simulink model "HSBI_Pedelec_Model"  (R2021b)
settings: Solver=ode4  StartTime=0.0  StopTime=t_end  FixedStep=t_step  RelTol=1e-3
values from neighbouring files (symbols this model uses):
  alphaGPX = [0 0 0 1.42108547152e-15 -7.50851856107e-05 -0.00056616369873 -0.00139814962361 -0.00223013361289 -0.00306211451479 -0.00389802874828 -0.00474974145994 -0.00561331371735 ... (6687 elements, 6687x1)]    [GPX_Simulink_Profil.mat]    (also in HSBI_Pedelec_Analyse_2.m = double(profil.alphaGPX(:)))
  c_R = 0.006    [HSBI_Pedelec_Parameter.m]
  c_w_A = 0.60    (= 0.6)    [HSBI_Pedelec_Parameter.m]
  E_Batt_nom = 500    [HSBI_Pedelec_Parameter.m]
  eta_G = 0.90    (= 0.9)    [HSBI_Pedelec_Parameter.m]
  eta_M = 0.80    (= 0.8)    [HSBI_Pedelec_Parameter.m]
  g = 9.81    [HSBI_Pedelec_Parameter.m]
  i_1 = 8    [HSBI_Pedelec_Parameter.m]
  i_2 = 5    [HSBI_Pedelec_Parameter.m]
  m = 135    [HSBI_Pedelec_Parameter.m]
  M_M_max = 5    [HSBI_Pedelec_Parameter.m]
  omega_M_max = 115    [HSBI_Pedelec_Parameter.m]
  P_F = 100    [HSBI_Pedelec_Parameter.m]
  P_M_max = 500    [HSBI_Pedelec_Parameter.m]
  r = 0.35    [HSBI_Pedelec_Parameter.m]
  rho = 1.225    [HSBI_Pedelec_Parameter.m]
  sGPX = [0 10 20 30 40 50 60 70 80 90 100 110 ... (6687 elements, 6687x1)]    [GPX_Simulink_Profil.mat]    (also in HSBI_Pedelec_Analyse_2.m = double(profil.sGPX(:)))
  SoC_0 = 1.00    (= 1)    [HSBI_Pedelec_Parameter.m]
  v_0 = 0    [HSBI_Pedelec_Analyse_2.m]
  v_fade = 23    [HSBI_Pedelec_Parameter.m]
  v_gs = 15    [HSBI_Pedelec_Parameter.m]
  v_max = 25    [HSBI_Pedelec_Parameter.m]
  v_min = 0.5    [HSBI_Pedelec_Parameter.m]
  x_0 = 0    [HSBI_Pedelec_Analyse_2.m]
settings Model: Creator=simon  LastModifiedBy=simon

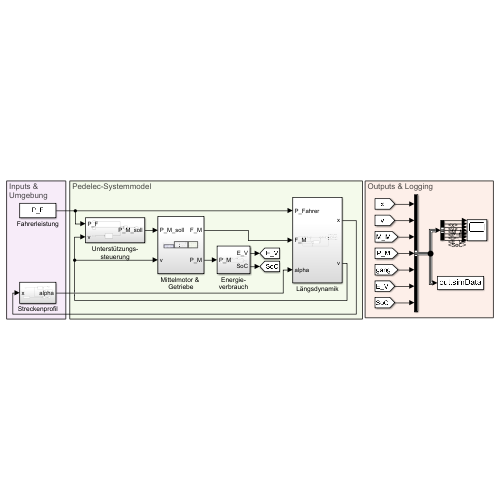
[thumbnail: Simulink's stored preview of the top-level diagram]
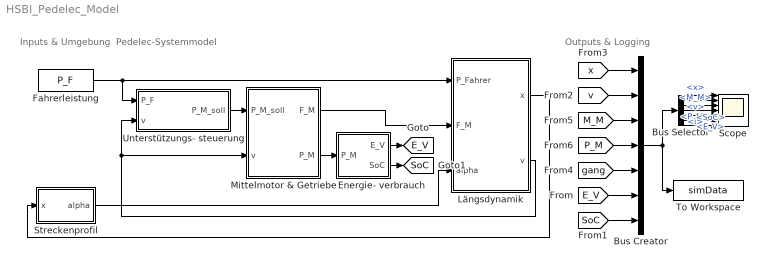
== system HSBI_Pedelec_Model ==
  note: Outputs & Logging
  note: Pedelec-Systemmodel
  note: Inputs &
      | Umgebung
  Bus Creator : BusCreator  Inputs=7
  Bus Selector : BusSelector  OutputSignals=x,v,M_M,P_M,i,E_V,SoC
  Energie- verbrauch : Subsystem
  Fahrerleistung : Constant  Value=P_F
  Längsdynamik : Subsystem
  Mittelmotor & Getriebe : Subsystem
  Scope : Scope  NumInputPorts=7
  Streckenprofil : Subsystem
  To Workspace : ToWorkspace  VariableName=simData  SaveFormat=Timeseries  SampleTime=-1
  Unterstützungs- steuerung : Subsystem
  tag scope: E_V=global, SoC=global
  wires:
  Mittelmotor & Getriebe/2(P_M) -> Energie- verbrauch/1(P_M)
  Fahrerleistung/1 -> Längsdynamik/1(P_Fahrer), Unterstützungs- steuerung/1(P_F)
  Streckenprofil/1(alpha) -> Längsdynamik/3(alpha)
  Längsdynamik/1(x) -> Streckenprofil/1(x)
  Längsdynamik/2(v) -> Unterstützungs- steuerung/2(v), Mittelmotor & Getriebe/2(v)
  Mittelmotor & Getriebe/1(F_M) -> Längsdynamik/2(F_M)
  Unterstützungs- steuerung/1(P_M_soll) -> Mittelmotor & Getriebe/1(P_M_soll)
  Energie- verbrauch/1(E_V) -> [E_V]
  Energie- verbrauch/2(SoC) -> [SoC]
  [M_M] -> Bus Creator/3
  [P_M] -> Bus Creator/4
  [gang] -> Bus Creator/5
  [x] -> Bus Creator/1
  [v] -> Bus Creator/2
  [E_V] -> Bus Creator/6
  [SoC] -> Bus Creator/7
  Bus Creator/1 -> Bus Selector/1, To Workspace/1
  Bus Selector/1 -> Scope/1  "<x>"
  Bus Selector/2 -> Scope/2  "<v>"
  Bus Selector/3 -> Scope/3  "<M_M>"
  Bus Selector/4 -> Scope/4  "<P_M>"
  Bus Selector/5 -> Scope/5  "<i>"
  Bus Selector/6 -> Scope/6  "<E_V>"
  Bus Selector/7 -> Scope/7  "<SoC>"

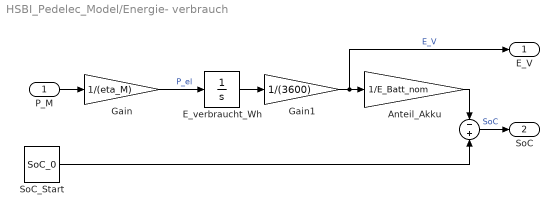
== system HSBI_Pedelec_Model/Energie- verbrauch ==
  P_M : Inport
  " " : Sum  Inputs=-+
  Anteil_Akku : Gain  Gain=1/E_Batt_nom
  E_verbraucht_Wh : Integrator
  Gain : Gain  Gain=1/(eta_M)
  Gain1 : Gain  Gain=1/(3600)
  SoC_Start : Constant  Value=SoC_0
  E_V : Outport
  SoC : Outport  Port=2
  wires:
  " "/1 -> SoC/1  "SoC"
  E_verbraucht_Wh/1 -> Gain1/1
  SoC_Start/1 -> " "/2
  Anteil_Akku/1 -> " "/1
  P_M/1 -> Gain/1
  Gain/1 -> E_verbraucht_Wh/1  "P_el"
  Gain1/1 -> E_V/1, Anteil_Akku/1  "E_V"

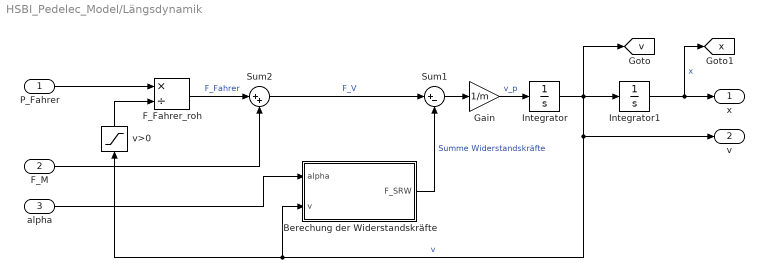
== system HSBI_Pedelec_Model/Längsdynamik ==
  P_Fahrer : Inport
  F_M : Inport  Port=2
  alpha : Inport  Port=3
  Berechung der Widerstandskräfte : MATLAB Function  TreatAsAtomicUnit=on
  F_Fahrer_roh : Product  Inputs=*/
  Gain : Gain  Gain=1/m
  Integrator : Integrator  InitialCondition=v_0
  Integrator1 : Integrator  InitialCondition=x_0
  Sum1 : Sum  Inputs=|+-
  Sum2 : Sum  Inputs=|++
  v>0 : Saturate  UpperLimit=inf  LowerLimit=v_min
  x : Outport
  v : Outport  Port=2
  tag scope: v=global, x=global
  wires:
  Sum2/1 -> Sum1/1  "F_V"
  Gain/1 -> Integrator/1  "v_p"
  Integrator/1 -> [v], Integrator1/1, v>0/1, Berechung der Widerstandskräfte/2(v), v/1  "v"
  Sum1/1 -> Gain/1
  alpha/1 -> Berechung der Widerstandskräfte/1(alpha)
  Integrator1/1 -> [x], x/1  "x"
  F_Fahrer_roh/1 -> Sum2/1  "F_Fahrer"
  Berechung der Widerstandskräfte/1(F_SRW) -> Sum1/2  "Summe Widerstandskräfte"
  v>0/1 -> F_Fahrer_roh/2
  F_M/1 -> Sum2/2
  P_Fahrer/1 -> F_Fahrer_roh/1

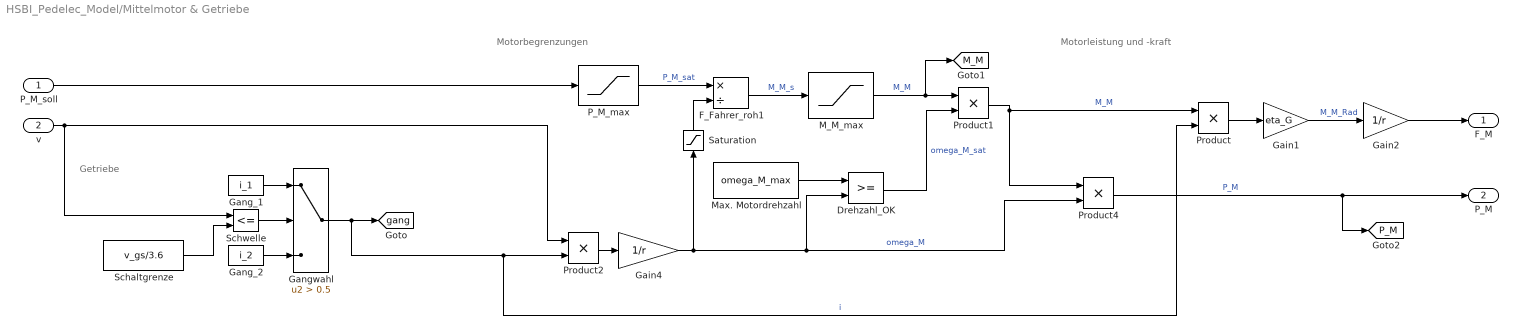
== system HSBI_Pedelec_Model/Mittelmotor & Getriebe ==
  note: Motorleistung und -kraft
  note: Motorbegrenzungen
  note: Getriebe
  P_M_soll : Inport
  v : Inport  Port=2
  Drehzahl_OK : RelationalOperator  OutDataTypeStr=boolean  RndMeth=Simplest
  F_Fahrer_roh1 : Product  Inputs=*/
  Gain1 : Gain  Gain=eta_G
  Gain2 : Gain  Gain=1/r
  Gain4 : Gain  Gain=1/r
  Gang_1 : Constant  Value=i_1
  Gang_2 : Constant  Value=i_2
  Gangwahl : Switch  Criteria=u2 > Threshold  Threshold=0.5
  M_M_max : Saturate  UpperLimit=M_M_max  LowerLimit=0
  Max. Motordrehzahl : Constant  Value=omega_M_max
  P_M_max : Saturate  UpperLimit=P_M_max  LowerLimit=0
  Product{,1..2,4} (4 alike) : Product
  Saturation : Saturate  UpperLimit=inf  LowerLimit=0.1
  Schaltgrenze : Constant  Value=v_gs/3.6
  Schwelle : RelationalOperator  Operator=<=  OutDataTypeStr=boolean  RndMeth=Simplest
  F_M : Outport
  P_M : Outport  Port=2
  tag scope: M_M=global, P_M=global, gang=global
  wires:
  Gain4/1 -> Drehzahl_OK/2, Product4/2, Saturation/1  "omega_M"
  M_M_max/1 -> [M_M], Product1/1  "M_M"
  Schwelle/1 -> Gangwahl/2
  Gangwahl/1 -> [gang], Product/2, Product2/2  "i"
  Product4/1 -> [P_M], P_M/1  "P_M"
  Gain1/1 -> Gain2/1  "M_M_Rad"
  Product1/1 -> Product4/1, Product/1  "M_M"
  Max. Motordrehzahl/1 -> Drehzahl_OK/1
  P_M_max/1 -> F_Fahrer_roh1/1  "P_M_sat"
  Drehzahl_OK/1 -> Product1/2  "omega_M_sat"
  Product2/1 -> Gain4/1
  F_Fahrer_roh1/1 -> M_M_max/1  "M_M_s"
  Product/1 -> Gain1/1
  Gang_1/1 -> Gangwahl/1
  Schaltgrenze/1 -> Schwelle/2
  Gain2/1 -> F_M/1
  P_M_soll/1 -> P_M_max/1
  Saturation/1 -> F_Fahrer_roh1/2
  v/1 -> Schwelle/1, Product2/1
  Gang_2/1 -> Gangwahl/3

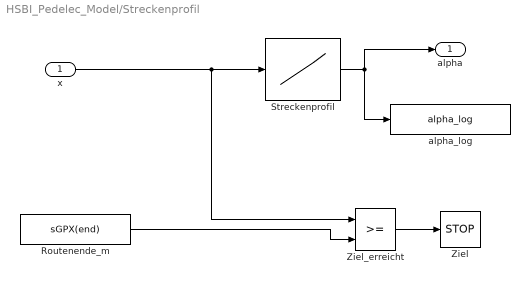
== system HSBI_Pedelec_Model/Streckenprofil ==
  x : Inport
  Routenende_m : Constant  Value=sGPX(end)
  Streckenprofil : Lookup_n-D  NumberOfTableDimensions=1  BreakpointsForDimension1=sGPX  Table=alphaGPX  InternalRulePriority=Speed  RndMeth=Simplest  InputSameDT=on
  Ziel : Stop
  Ziel_erreicht : RelationalOperator  OutDataTypeStr=boolean  RndMeth=Simplest
  alpha_log : ToWorkspace  VariableName=alpha_log  SaveFormat=Timeseries  SampleTime=-1
  alpha : Outport
  wires:
  Streckenprofil/1 -> alpha/1, alpha_log/1
  x/1 -> Ziel_erreicht/1, Streckenprofil/1
  Routenende_m/1 -> Ziel_erreicht/2
  Ziel_erreicht/1 -> Ziel/1

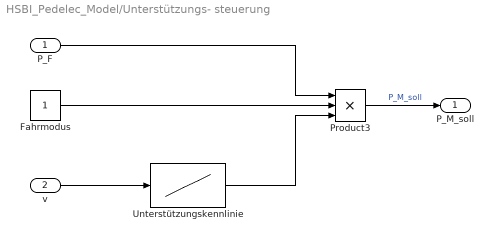
== system HSBI_Pedelec_Model/Unterstützungs- steuerung ==
  P_F : Inport
  v : Inport  Port=2
  Fahrmodus : Constant
  Product3 : Product  Inputs=3
  Unterstützungskennlinie : Lookup_n-D  NumberOfTableDimensions=1  BreakpointsForDimension1=[0 v_fade/3.6 v_max/3.6]  Table=[1 1 0]  ExtrapMethod=Clip  InternalRulePriority=Speed  RndMeth=Simplest  InputSameDT=on
  P_M_soll : Outport
  wires:
  Fahrmodus/1 -> Product3/2
  v/1 -> Unterstützungskennlinie/1
  Product3/1 -> P_M_soll/1  "P_M_soll"
  Unterstützungskennlinie/1 -> Product3/3
  P_F/1 -> Product3/1

== matlab function HSBI_Pedelec_Model/Längsdynamik/Berechung der Widerstandskräfte ==
  data: alpha input; F_SRW output; v input; m parameter; g parameter; c_R parameter; rho parameter; c_w_A parameter
function F_SRW= fcn(alpha, v, m, g, c_R, rho, c_w_A)

F_S = m*g*sin(alpha);
F_R = c_R*m*g*cos(alpha);
F_W = 0.5*rho*c_w_A*v^2;
F_SRW = F_S+F_R+F_W;
